simulink subsystem "Robot_Control_sub"  (R2023b)
settings: Solver=VariableStepAuto  StartTime=0.0  StopTime=10.0  RelTol=1e-3
undefined symbols (not defined in the file): ballMotor_Set_Desiredspeed, HoodServo_Position
libraries: simulink x1, Controls_Components_lib x1
settings Model: Creator=USER  LastModifiedBy=ander

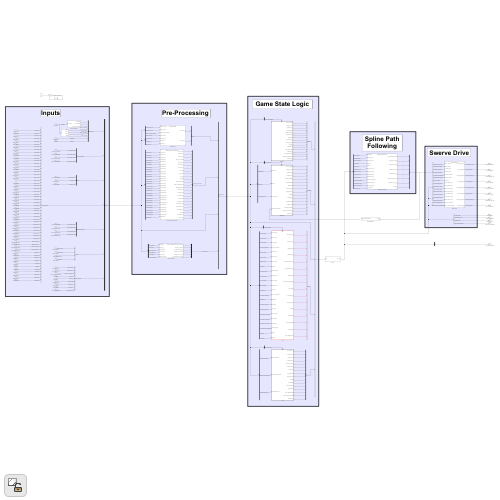
[thumbnail: Simulink's stored preview of the top-level diagram]
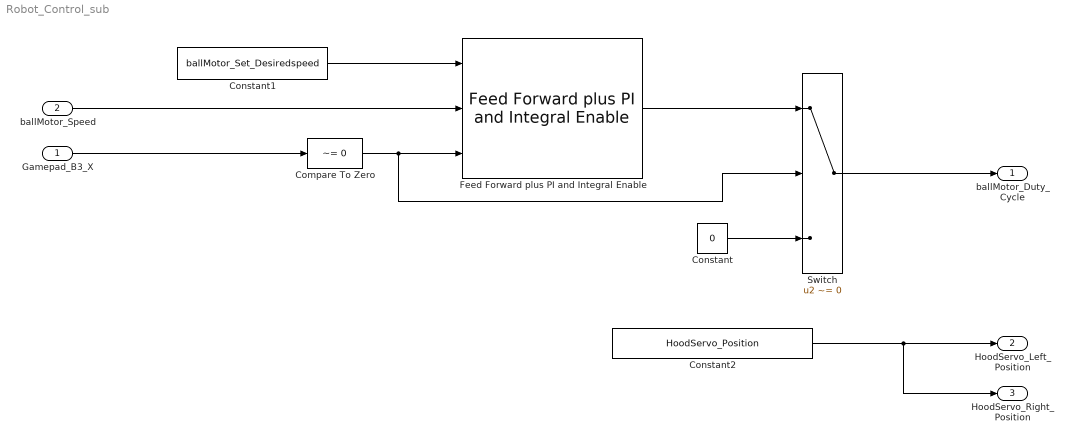
== system Robot_Control_sub ==
  Gamepad_B3_X : Inport
  ballMotor_Speed : Inport  Port=2
  Compare To Zero : simulink/Logic and Bit Operations/Compare To Zero  relop=~=  OutDataTypeStr=boolean
  Constant : Constant  Value=0
  Constant1 : Constant  Value=ballMotor_Set_Desiredspeed
  Constant2 : Constant  Value=HoodServo_Position
  Feed Forward plus PI and Integral Enable : Controls_Components_lib/Feed Forward plus PI and Integral Enable  Gain_FF=Ballmotor_speed_Kff  Gain_P=Ballmotor_speed_Kp  Gain_I=Ballmotor_speed_Ki  Limit_I_Upper=0.1  Limit_I_Lower=-0.1  Limit_T_Upper=1  Limit_T_Lower=0
  Switch : Switch  Criteria=u2 ~= 0  SaturateOnIntegerOverflow=off  InputSameDT=off
  ballMotor_Duty_Cycle : Outport
  HoodServo_Left_Position : Outport  Port=2
  HoodServo_Right_Position : Outport  Port=3
  wires:
  Constant/1 -> Switch/3
  Switch/1 -> ballMotor_Duty_Cycle/1
  Gamepad_B3_X/1 -> Compare To Zero/1
  Feed Forward plus PI and Integral Enable/1 -> Switch/1
  Constant1/1 -> Feed Forward plus PI and Integral Enable/1
  ballMotor_Speed/1 -> Feed Forward plus PI and Integral Enable/2
  Compare To Zero/1 -> Feed Forward plus PI and Integral Enable/3, Switch/2
  Constant2/1 -> HoodServo_Left_Position/1, HoodServo_Right_Position/1
